simulink model "linear_decoupling_model"  (R2024b)
settings: Solver=ode4  StartTime=0.0  StopTime=150  FixedStep=0.001  RelTol=1e-3
PreLoadFcn:
  | run('JacobianAnalysis.m')
InitFcn:
  | run('JacobianAnalysis.m')
values from neighbouring files (symbols this model uses):
  A1_analysis = double(A1_analysis)    [JacobianAnalysis.m]
  A2_analysis = double(A2_analysis)    [JacobianAnalysis.m]
  B1_analysis = double(B1_analysis)    [JacobianAnalysis.m]
  B2_analysis = double(B2_analysis)    [JacobianAnalysis.m]
  X0 = [op_trim3.States(1, 1).x;op_trim3.States(2,1).x;op_trim3.States(3,1).x;op_trim3.States(4,1).x]    [JacobianAnalysis.m]
settings Model: Creator=LocoalKOH  LastModifiedBy=LocoalKOH

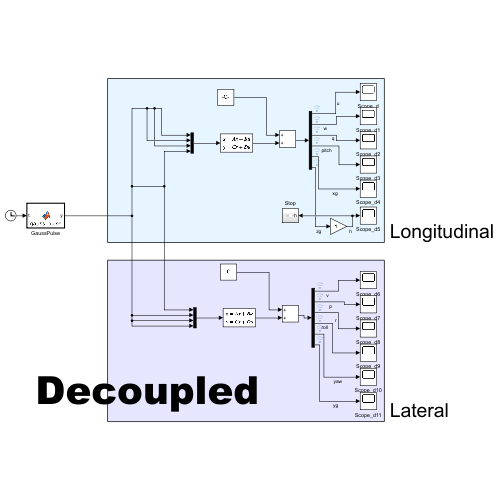
[thumbnail: Simulink's stored preview of the top-level diagram]
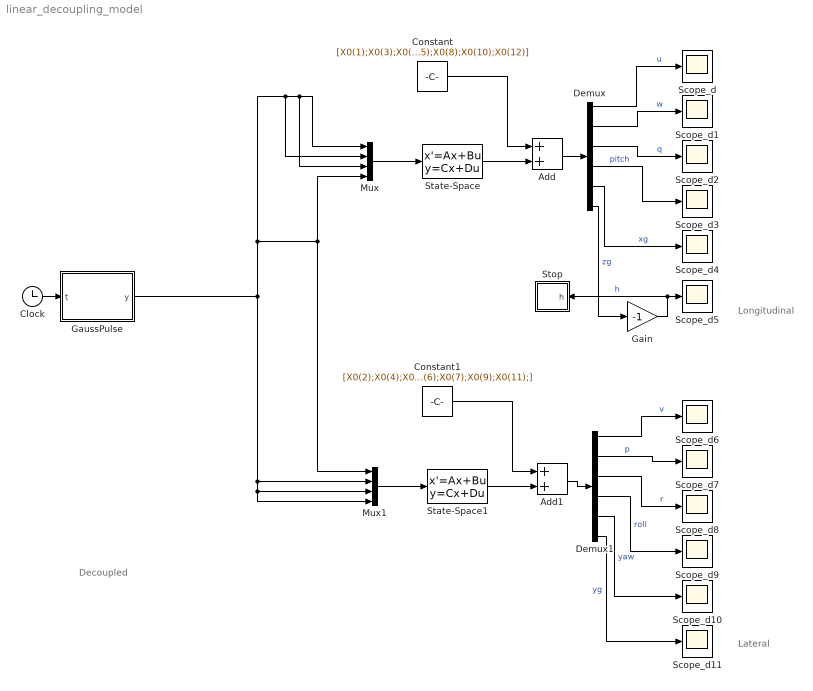
== system linear_decoupling_model ==
  note: Longitudinal
  note: Decoupled
  note: Lateral
  Add : Sum
  Add1 : Sum
  Clock : Clock
  Constant : Constant  Value=[X0(1);X0(3);X0(5);X0(8);X0(10);X0(12)]  VectorParams1D=off
  Constant1 : Constant  Value=[X0(2);X0(4);X0(6);X0(7);X0(9);X0(11);]  VectorParams1D=off
  Demux : Demux  Outputs=6
  Demux1 : Demux  Outputs=6
  Gain : Gain  Gain=-1
  GaussPulse : MATLAB Function  TreatAsAtomicUnit=on
  Mux : Mux
  Mux1 : Mux
  Scope_d{,1..11} (12 alike) : Scope
  State-Space : StateSpace  A=A1_analysis  B=B1_analysis  C=eye(6)  D=zeros(6,4)  InitialCondition=zeros(6,1)  ContinuousStateAttributes={'u','w','q','pitch','xg','zg'}
  State-Space1 : StateSpace  A=A2_analysis  B=B2_analysis  C=eye(6)  D=zeros(6,4)  InitialCondition=zeros(6,1)  ContinuousStateAttributes={'v','p','r','yaw','yg','roll'}
  Stop : Subsystem
  wires:
  Mux/1 -> State-Space/1
  Demux/1 -> Scope_d/1  "u"
  Demux/2 -> Scope_d1/1  "w"
  Demux/3 -> Scope_d2/1  "q"
  Demux/4 -> Scope_d3/1  "pitch"
  State-Space/1 -> Add/2
  Add/1 -> Demux/1
  Constant/1 -> Add/1
  Demux1/2 -> Scope_d7/1  "p"
  Mux1/1 -> State-Space1/1
  Demux1/1 -> Scope_d6/1  "v"
  State-Space1/1 -> Add1/2
  Add1/1 -> Demux1/1
  Constant1/1 -> Add1/1
  GaussPulse/1(y) -> Mux/3, Mux/1, Mux/2, Mux1/1, Mux/4, Mux1/4, Mux1/3, Mux1/2
  Demux1/4 -> Scope_d9/1  "roll"
  Demux1/3 -> Scope_d8/1  "r"
  Gain/1 -> Stop/1(h), Scope_d5/1  "h"
  Clock/1 -> GaussPulse/1(t)
  Demux/6 -> Gain/1  "zg"
  Demux1/5 -> Scope_d10/1  "yaw"
  Demux1/6 -> Scope_d11/1  "yg"
  Demux/5 -> Scope_d4/1  "xg"

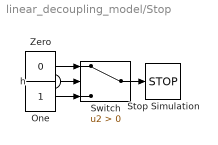
== system linear_decoupling_model/Stop ==
  h : Inport
  One : Constant  OutDataTypeStr=Inherit: Inherit via back propagation
  Stop Simulation : Stop
  Switch : Switch  Criteria=u2 > Threshold  SaturateOnIntegerOverflow=off  InputSameDT=off
  Zero : Constant  Value=0  OutDataTypeStr=Inherit: Inherit via back propagation
  wires:
  One/1 -> Switch/3
  Zero/1 -> Switch/1
  Switch/1 -> Stop Simulation/1
  h/1 -> Switch/2

== matlab function linear_decoupling_model/GaussPulse ==
  data: t input; y output
function y = gauss_pulse(t)
    y = 0.1 * exp(-(t - 5)^2 / 0.1);  % 在t=5秒附近有扰动
end
